simulink model "three_phase_dab"  (R2026a)
settings: Solver=ode23tb  StopTime=param.sim.simlength  FixedStep=tc  MaxStep=param.glb_time.tc
values from neighbouring files (symbols this model uses):
  param = struct()    [init_model.m]
libraries: fl_lib x30, nesl_utility x23, discrete_time_low_pass_filter x6, single_phase_transformer x3, lithium_ion_battery x2, pi_ctrl x2, three_phase_inverter_ideal_switch_based_model x2, three_phase_inverter_mosfet_based_with_thermal_model x2, three_phase_dab_modulator x1
(part 1 of 2)
settings Model: SimulationMode=accelerator  Creator=LTNBDA  LastModifiedBy=dbagn
settings SolverCC: ZeroCrossControl=EnableAll  ZeroCrossAlgorithm=Adaptive  SolverResetMethod=Robust
settings DataIOCC: MaxDataPoints=1  SignalLoggingSaveFormat=ModelDataLogs
settings OptimizationCC: InitFltsAndDblsToZero=on  EfficientMapNaN2IntZero=off
settings DebuggingCC: SaveWithParameterizedLinksMsg=none  SignalResolutionControl=TryResolveAllWithWarning  MultiTaskDSMMsg=warning  MultiTaskCondExecSysMsg=none  MultiTaskRateTransMsg=warning
settings HardwareCC: ProdBitPerLong=64.0  ProdHWDeviceType=Generic->64-bit Embedded Processor (LP64)  TargetBitPerPointer=64.0  TargetBitPerSizeT=64.0  TargetBitPerPtrDiffT=64.0  TargetLongLongMode=on  TargetIntDivRoundTo=Zero  TargetEndianess=LittleEndian  TargetWordSize=64.0  TargetHWDeviceType=MATLAB Host  ProdEqTarget=off
settings SFSimCC: SimCustomHeaderCode=|
  | #include "rpi.h"
  | #include "rpi_simulink.h"
  | #include "mavgflt.h"
  | #include "mavgflt_simulink.h"
  | #include "mavgflts.h"
  | #include "mavgflts_simulink.h"
  | #include "dsmavgflt.h"
  | #include "dsmavgflt_simulink.h"
  | #include "bemf_obsv.h"
  | #include "bemf_obsv_simulink.h"
  | #include "bemf_obsv_load_est.h"
  | #include "bemf_obsv_load_est_simulink.h"
  | #include "dqvector_pi.h"
  | #include "dqvector_pi_simulink.h"
  | #include "sv_pwm_simulink.h"
  | #include "sv_pwm.h"
  | #include "first_harmonic_tracker.h"
  | #include "first_harmonic_tracker_simulink.h"
  | #include "dqpll_thyr.h"
  | #include "dqpll_thyr_simulink.h"
  | #include "dqpll_grid.h"
  | #include "dqpll_grid_simulink.h"
  | #include "linear_double_integrator_observer_simulink.h"
  | #include "linear_double_integrator_observer.h"
  | #include "sv_pwm_cm_simulink.h"
  | #include "sv_pwm_cm.h"
settings SFSimCC: SimUserSources=|
  | "rpi.c"
  | "rpi_simulink.c"
  | "mavgflt_simulink.c"
  | "mavgflt.c"
  | "mavgflts_simulink.c"
  | "mavgflts.c"
  | "dsmavgflt_simulink.c"
  | "dsmavgflt.c"
  | "bemf_obsv_simulink.c"
  | "bemf_obsv.c"
  | "bemf_obsv_load_est_simulink.c"
  | "bemf_obsv_load_est.c"
  | "dqvector_pi.c"
  | "dqvector_pi_simulink.c"
  | "sv_pwm_simulink.c"
  | "sv_pwm.c"
  | "first_harmonic_tracker_simulink.c"
  | "first_harmonic_tracker.c"
  | "dqpll_thyr_simulink.c"
  | "dqpll_thyr.c"
  | "dqpll_grid_simulink.c"
  | "dqpll_grid.c"
  | "linear_double_integrator_observer_simulink.c"
  | "linear_double_integrator_observer.c"
  | "sv_pwm_cm_simulink.c"
  | "sv_pwm_cm.c"
settings SFSimCC: SimUserIncludeDirs=|
  | include
  | src
settings CodeAppCC: MaxIdLength=128.0
settings GRTTargetCC: CombineOutputUpdateFcns=off  GRTInterface=on
settings SimscapeCC: SimscapeNormalizeSystem=off  SimscapeNominalValues="[{\"value\":\"1\",\"unit\":\"A\"},{\"value\":\"1\",\"unit\":\"bar\"},{\"value\":\"1\",\"unit\":\"cm^2\"},{\"value\":\"1\",\"unit\":\"cm^3/s\"},{\"value\":\"1\",\"unit\":\"kJ/kg\"},{\"value\":\"1\",\"unit\":\"kW\"},{\"value\":\"1\",\"unit\":\"l\"},{\"value\":\"1\",\"unit\":\"N\"},{\"value\":\"1\",\"unit\":\"N*m\"},{\"value\":\"1\",\"unit\":\"V\"}]"  SimscapeLogType=none  SimscapeLogDataHistory=5000.0

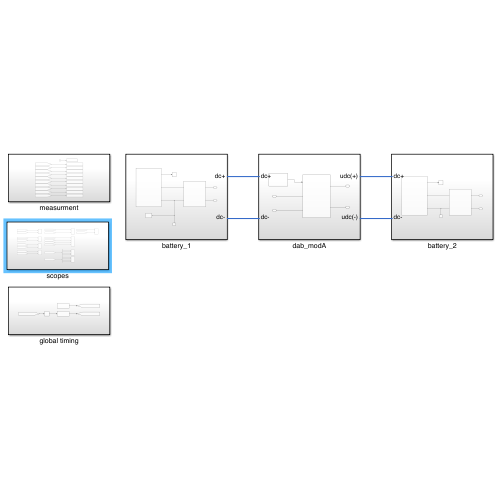
[thumbnail: Simulink's stored preview of the top-level diagram]
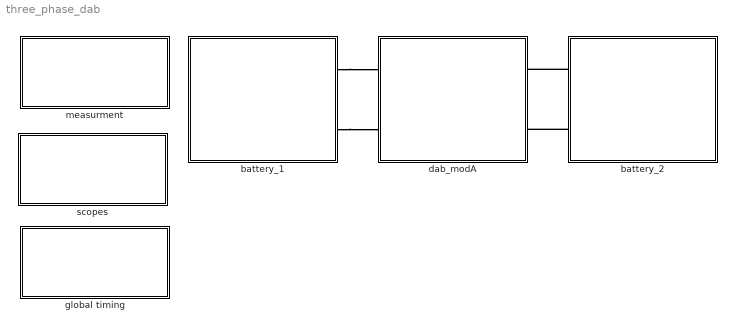
== system three_phase_dab ==
  battery_1 : Subsystem
  battery_2 : Subsystem
  dab_modA : Subsystem
  global timing : Subsystem
  measurment : Subsystem
  scopes : Subsystem
  connections:
  battery_2/RConn2 -- dab_modA/RConn2
  battery_2/RConn1 -- dab_modA/RConn1
  battery_1/RConn1 -- dab_modA/LConn1
  battery_1/RConn2 -- dab_modA/LConn2

== system three_phase_dab/battery_1 ==
  Electrical Reference1 : fl_lib/Electrical/Electrical Elements/Electrical Reference
  Solver Configuration : nesl_utility/Solver Configuration  PhysicalDomain=network_engine_domain  SubClassName=solver  LeftPortType=input  RightPortType=generic  Tones=[]  Harmonics=[]  SimulateNoise=off  Profile=off  UseLocalSampling=off  EnableSwitchedLinearOptims=on  FrequencyDomain=off  UseCCode=off  RelTol=0.001  AbsTol=0.001  MinStep=1e-09  ToWorkspace=off  RevertToSquareIcSolve=off  NumHomotopyIterations=100  PhasorMode=off  PhasorModeNumHarmonics=1  ConsistencySolver=NEWTON_FTOL  CanonicalOrdering=UNORDERED  OptimizeIntermediates=UNOPTIMIZED  IndexReductionMethod=DerivativeReplacement  DoDC=on  ResidualTolerance=1e-3  ConsistencyTolSource=GLOBAL  ConsistencyAbsTol=0.001  ConsistencyRelTol=0.001  ConsistencyTolFactor=0.001  UseLocalSolver=on  LocalSolverChoice=NE_BACKWARD_EULER_ADVANCER  ResolveIndetEquations=on  FunctionEvalNumThread=1  LocalSolverSampleTime=param.glb_time.tc  DoFixedCost=on  MaxNonlinIter=param.sim.nonlinear_iterations  MaxModeIter=2  ComputeImpulses=off  ImpulseIterations=2  LinearAlgebra=auto  LinearAlgebraNumThread=0  EquationFormulation=NE_TIME_EF  DelaysMemoryBudget=1024  AutomaticFiltering=on  FilteringTimeConstant=0.001  PartitionStorageMethod=AS_NEEDED  PartitionMemoryBudget=1024  PartitionMethod=ROBUST  MultibodyUseLocalSolver=off  MultibodyLocalSolverChoice=ODE1  MultibodyLocalSolverSampleTime=0.001
  lithium ion battery 1 : Scope
      settings: ActiveDisplayYMinimum=-6265.3075005586525  ActiveDisplayYMaximum=7146.6490040654116  DataLoggingVariableName=ScopeData3
  lithium_ion_battery : lithium_ion_battery/lithium_ion_battery  Q=param.battery.pack_1.Q  number_of_cells=param.battery.pack_1.number_of_cells  E_1=param.battery.pack_1.E_1  E0=param.battery.pack_1.E0  E1=param.battery.pack_1.E1  E2=param.battery.pack_1.E2  E3=param.battery.pack_1.E3  Elog=param.battery.pack_1.Elog  R0=param.battery.pack_1.R0  R1=param.battery.pack_1.R1  C1=param.battery.pack_1.C1  M=param.battery.pack_1.M  alpha=param.battery.pack_1.alpha  soc_init=param.battery.pack_1.soc_init  ts_battery=param.glb_time.ts_dab  q1Kalman=param.battery.pack_1.q1Kalman  q2Kalman=param.battery.pack_1.q2Kalman  q3Kalman=param.battery.pack_1.q3Kalman  rKalman=param.battery.pack_1.rKalman  tc=param.glb_time.tc  battery_voltage_init_m=param.battery.ocv_1
  single_phase_ui_measure : Subsystem
  dc+ : PMIOPort  Side=Right
  dc- : PMIOPort  Port=2  Side=Right
  wires:
  lithium_ion_battery/1 -> lithium ion battery 1/1
  connections:
  single_phase_ui_measure/LConn2 -- lithium_ion_battery/RConn2 -- Electrical Reference1/LConn1 -- Solver Configuration/RConn1
  single_phase_ui_measure/RConn1 -- dc+/RConn1
  lithium_ion_battery/RConn1 -- single_phase_ui_measure/LConn1
  dc-/RConn1 -- single_phase_ui_measure/RConn2

== system three_phase_dab/battery_2 ==
  Electrical Reference1 : fl_lib/Electrical/Electrical Elements/Electrical Reference
  lithium ion battery 2 : Scope
      settings: ActiveDisplayYMinimum=-4779.68523514888  ActiveDisplayYMaximum=38953.418417165572  DataLoggingVariableName=ScopeData3
  lithium_ion_battery : lithium_ion_battery/lithium_ion_battery  Q=param.battery.pack_2.Q  number_of_cells=param.battery.pack_2.number_of_cells  E_1=param.battery.pack_2.E_1  E0=param.battery.pack_2.E0  E1=param.battery.pack_2.E1  E2=param.battery.pack_2.E2  E3=param.battery.pack_2.E3  Elog=param.battery.pack_2.Elog  R0=param.battery.pack_2.R0  R1=param.battery.pack_2.R1  C1=param.battery.pack_2.C1  M=param.battery.pack_2.M  alpha=param.battery.pack_2.alpha  soc_init=param.battery.pack_2.soc_init  ts_battery=param.glb_time.ts_dab  q1Kalman=param.battery.pack_2.q1Kalman  q2Kalman=param.battery.pack_2.q2Kalman  q3Kalman=param.battery.pack_2.q3Kalman  rKalman=param.battery.pack_2.rKalman  tc=param.glb_time.tc  battery_voltage_init_m=param.battery.ocv_2
  single_phase_ui_measure : Subsystem
  dc+ : PMIOPort  Side=Right
  dc- : PMIOPort  Port=2  Side=Right
  wires:
  lithium_ion_battery/1 -> lithium ion battery 2/1
  connections:
  dc-/RConn1 -- single_phase_ui_measure/RConn2
  lithium_ion_battery/RConn1 -- single_phase_ui_measure/LConn1
  single_phase_ui_measure/RConn1 -- dc+/RConn1
  Electrical Reference1/LConn1 -- lithium_ion_battery/RConn2 -- single_phase_ui_measure/LConn2

== system three_phase_dab/dab_modA ==
  dab_ctrl : Subsystem
  dcdc_with_galvanic_isolation : Subsystem
  udc(+) : PMIOPort  Side=Right
  udc(-) : PMIOPort  Port=2  Side=Right
  dc+ : PMIOPort  Port=3  Side=Left
  dc- : PMIOPort  Port=4  Side=Left
  wires:
  dab_ctrl/1(gate_cmds) -> dcdc_with_galvanic_isolation/1(gate_cmds)
  connections:
  udc(+)/RConn1 -- dcdc_with_galvanic_isolation/RConn1
  udc(-)/RConn1 -- dcdc_with_galvanic_isolation/RConn2
  dc-/RConn1 -- dcdc_with_galvanic_isolation/LConn2
  dc+/RConn1 -- dcdc_with_galvanic_isolation/LConn1

== system three_phase_dab/global timing ==
  Unit Delay : UnitDelay  SampleTime=param.glb_time.tc
  time_afe1 : Subsystem  mask{k=1}
      mask prompts: k "Time Gain"
      mask Display:
      | disp('time-gen');
      | port_label('input', 1, 'crt');
      | port_label('output', 1, 'tout');
  time_afe3 : Subsystem  mask{k=1}
      mask prompts: k "Time Gain"
      mask Display:
      | disp('time-gen');
      | port_label('output', 1, 'tout');
  tag scope: time_dab_module_1=global, time_master=global
  wires:
  time_afe1/1(Out1) -> [time_dab_module_1]
  time_afe3/1(Out1) -> [time_master]
  [local_time_corr_llc_mod1] -> Unit Delay/1
  Unit Delay/1 -> time_afe1/1(correction_time)

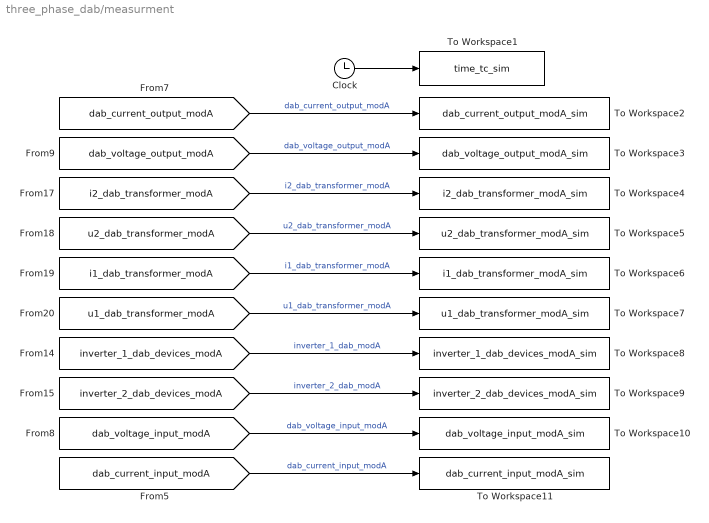
== system three_phase_dab/measurment ==
  Clock : Clock
  To Workspace1 : ToWorkspace  VariableName=time_tc_sim  SampleTime=param.glb_time.tc
      settings: MaxDataPoints=param.glb_time.Nc  Decimation=param.glb_time.decimation_tc
  To Workspace10 : ToWorkspace  VariableName=dab_voltage_input_modA_sim  SampleTime=param.glb_time.tc
      settings: MaxDataPoints=param.glb_time.Nc  Decimation=param.glb_time.decimation_tc
  To Workspace11 : ToWorkspace  VariableName=dab_current_input_modA_sim  SampleTime=param.glb_time.tc
      settings: MaxDataPoints=param.glb_time.Nc  Decimation=param.glb_time.decimation_tc
  To Workspace2 : ToWorkspace  VariableName=dab_current_output_modA_sim  SampleTime=param.glb_time.tc
      settings: MaxDataPoints=param.glb_time.Nc  Decimation=param.glb_time.decimation_tc
  To Workspace3 : ToWorkspace  VariableName=dab_voltage_output_modA_sim  SampleTime=param.glb_time.tc
      settings: MaxDataPoints=param.glb_time.Nc  Decimation=param.glb_time.decimation_tc
  To Workspace4 : ToWorkspace  VariableName=i2_dab_transformer_modA_sim  SampleTime=param.glb_time.tc
      settings: MaxDataPoints=param.glb_time.Nc  Decimation=param.glb_time.decimation_tc
  To Workspace5 : ToWorkspace  VariableName=u2_dab_transformer_modA_sim  SampleTime=param.glb_time.tc
      settings: MaxDataPoints=param.glb_time.Nc  Decimation=param.glb_time.decimation_tc
  To Workspace6 : ToWorkspace  VariableName=i1_dab_transformer_modA_sim  SampleTime=param.glb_time.tc
      settings: MaxDataPoints=param.glb_time.Nc  Decimation=param.glb_time.decimation_tc
  To Workspace7 : ToWorkspace  VariableName=u1_dab_transformer_modA_sim  SampleTime=param.glb_time.tc
      settings: MaxDataPoints=param.glb_time.Nc  Decimation=param.glb_time.decimation_tc
  To Workspace8 : ToWorkspace  VariableName=inverter_1_dab_devices_modA_sim  SampleTime=param.glb_time.tc
      settings: MaxDataPoints=param.glb_time.Nc  Decimation=param.glb_time.decimation_tc
  To Workspace9 : ToWorkspace  VariableName=inverter_2_dab_devices_modA_sim  SampleTime=param.glb_time.tc
      settings: MaxDataPoints=param.glb_time.Nc  Decimation=param.glb_time.decimation_tc
  wires:
  Clock/1 -> To Workspace1/1
  [dab_current_output_modA] -> To Workspace2/1  "dab_current_output_modA"
  [dab_voltage_output_modA] -> To Workspace3/1  "dab_voltage_output_modA"
  [i2_dab_transformer_modA] -> To Workspace4/1  "i2_dab_transformer_modA"
  [u1_dab_transformer_modA] -> To Workspace7/1  "u1_dab_transformer_modA"
  [i1_dab_transformer_modA] -> To Workspace6/1  "i1_dab_transformer_modA"
  [u2_dab_transformer_modA] -> To Workspace5/1  "u2_dab_transformer_modA"
  [inverter_1_dab_devices_modA] -> To Workspace8/1  "inverter_1_dab_modA"
  [inverter_2_dab_devices_modA] -> To Workspace9/1  "inverter_2_dab_modA"
  [dab_voltage_input_modA] -> To Workspace10/1  "dab_voltage_input_modA"
  [dab_current_input_modA] -> To Workspace11/1  "dab_current_input_modA"

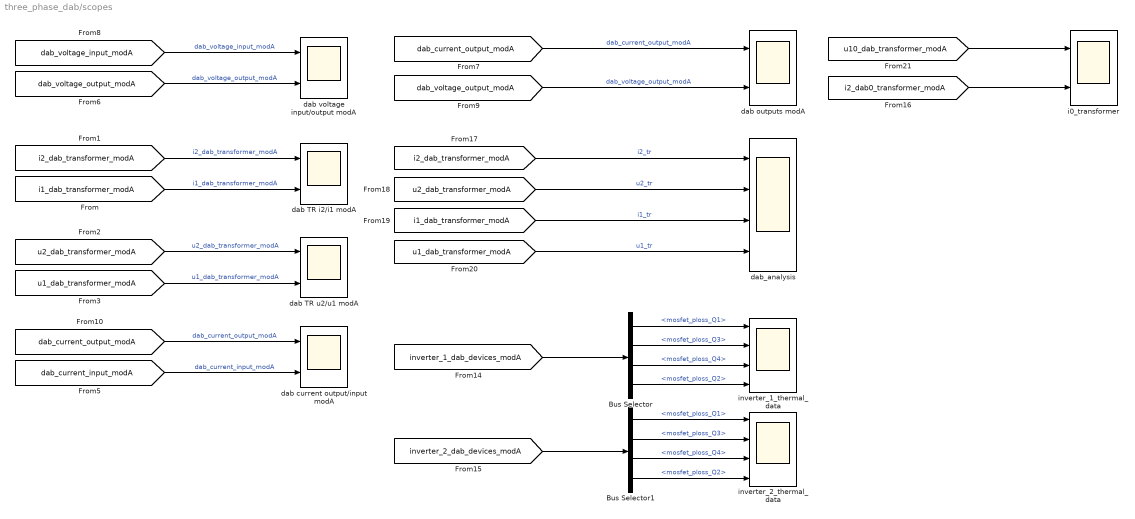
== system three_phase_dab/scopes ==
  Bus Selector : BusSelector  OutputSignals=mosfet_ploss_Q1,mosfet_ploss_Q3,mosfet_ploss_Q4,mosfet_ploss_Q2
  Bus Selector1 : BusSelector  OutputSignals=mosfet_ploss_Q1,mosfet_ploss_Q3,mosfet_ploss_Q4,mosfet_ploss_Q2
  dab TR i2/i1 modA : Scope  NumInputPorts=2
      settings: SampleTime=param.glb_time.tc  ActiveDisplayYMinimum=-2129.3112232140747  ActiveDisplayYMaximum=1620.3891398774613  DataLoggingVariableName=ScopeData13
  dab TR u2/u1 modA : Scope  NumInputPorts=2
      settings: SampleTime=param.glb_time.tc  ActiveDisplayYMinimum=-1578.7453878307324  ActiveDisplayYMaximum=1578.7340154658184  DataLoggingVariableName=ScopeData4
  dab current output/input modA : Scope  NumInputPorts=2
      settings: SampleTime=param.glb_time.tc  ActiveDisplayYMinimum=-1089.9608600530696  ActiveDisplayYMaximum=2070.2962931787843  DataLoggingVariableName=ScopeData8
  dab outputs modA : Scope  NumInputPorts=2
      settings: SampleTime=param.glb_time.tc  ActiveDisplayYMinimum=-644.40009841688664  ActiveDisplayYMaximum=609.5912225853051  DataLoggingVariableName=ScopeData6
  dab voltage input/output modA : Scope  NumInputPorts=2
      settings: SampleTime=param.glb_time.tc  ActiveDisplayYMinimum=1182.800968165963  ActiveDisplayYMaximum=1251.5348190400946  DataLoggingVariableName=ScopeData10
  dab_analysis : Scope  NumInputPorts=4
      settings: ActiveDisplayYMinimum=-934.40964830703967  ActiveDisplayYMaximum=936.03082553931858  DataLoggingVariableName=ScopeData14
  i0_transformer : Scope  NumInputPorts=2
      settings: SampleTime=param.glb_time.tc  ActiveDisplayYMinimum=-1.8947806286936003E-13  ActiveDisplayYMaximum=1.8947806286936003E-13  DataLoggingVariableName=ScopeData11
  inverter_1_thermal_data : Scope  NumInputPorts=4
      settings: SampleTime=param.glb_time.tc  ActiveDisplayYMinimum=-41.459984697896282  ActiveDisplayYMaximum=413.8102017159581
  inverter_2_thermal_data : Scope  NumInputPorts=4
      settings: SampleTime=param.glb_time.tc  ActiveDisplayYMinimum=-81.726801597383641  ActiveDisplayYMaximum=735.5412143764529  DataLoggingVariableName=ScopeData9
  wires:
  [dab_voltage_input_modA] -> dab voltage input/output modA/1  "dab_voltage_input_modA"
  [dab_current_output_modA] -> dab current output/input modA/1  "dab_current_output_modA"
  [dab_voltage_output_modA] -> dab voltage input/output modA/2  "dab_voltage_output_modA"
  [dab_current_input_modA] -> dab current output/input modA/2  "dab_current_input_modA"
  [i2_dab_transformer_modA] -> dab TR i2/i1 modA/1  "i2_dab_transformer_modA"
  [i1_dab_transformer_modA] -> dab TR i2/i1 modA/2  "i1_dab_transformer_modA"
  [u2_dab_transformer_modA] -> dab TR u2/u1 modA/1  "u2_dab_transformer_modA"
  [u1_dab_transformer_modA] -> dab TR u2/u1 modA/2  "u1_dab_transformer_modA"
  [dab_voltage_output_modA] -> dab outputs modA/2  "dab_voltage_output_modA"
  [dab_current_output_modA] -> dab outputs modA/1  "dab_current_output_modA"
  [inverter_1_dab_devices_modA] -> Bus Selector/1
  Bus Selector/1 -> inverter_1_thermal_data/1  "<mosfet_ploss_Q1>"
  Bus Selector/2 -> inverter_1_thermal_data/2  "<mosfet_ploss_Q3>"
  Bus Selector/3 -> inverter_1_thermal_data/3  "<mosfet_ploss_Q4>"
  Bus Selector/4 -> inverter_1_thermal_data/4  "<mosfet_ploss_Q2>"
  Bus Selector1/4 -> inverter_2_thermal_data/4  "<mosfet_ploss_Q2>"
  Bus Selector1/3 -> inverter_2_thermal_data/3  "<mosfet_ploss_Q4>"
  Bus Selector1/2 -> inverter_2_thermal_data/2  "<mosfet_ploss_Q3>"
  Bus Selector1/1 -> inverter_2_thermal_data/1  "<mosfet_ploss_Q1>"
  [inverter_2_dab_devices_modA] -> Bus Selector1/1
  [i2_dab0_transformer_modA] -> i0_transformer/2
  [u10_dab_transformer_modA] -> i0_transformer/1
  [u2_dab_transformer_modA] -> dab_analysis/2  "u2_tr"
  [i2_dab_transformer_modA] -> dab_analysis/1  "i2_tr"
  [u1_dab_transformer_modA] -> dab_analysis/4  "u1_tr"
  [i1_dab_transformer_modA] -> dab_analysis/3  "i1_tr"

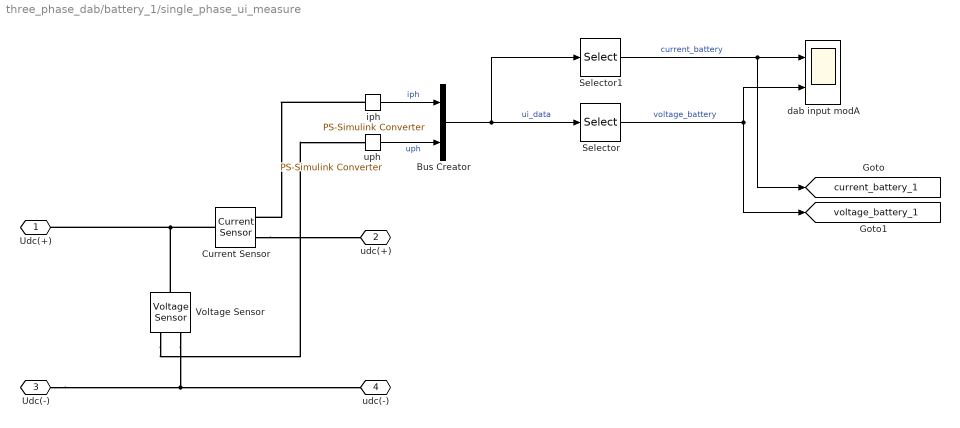
== system three_phase_dab/battery_1/single_phase_ui_measure ==
  Bus Creator : BusCreator  Inputs=2
  Current Sensor : fl_lib/Electrical/Electrical Sensors/Current Sensor
  Selector : Selector  InputPortWidth=2  IndexOptions=Index vector (dialog)  Indices=2  OutputSizes=1
  Selector1 : Selector  InputPortWidth=2  IndexOptions=Index vector (dialog)  Indices=1  OutputSizes=1
  Voltage Sensor : fl_lib/Electrical/Electrical Sensors/Voltage Sensor
  dab input modA : Scope  NumInputPorts=2
      settings: SampleTime=param.glb_time.tc  ActiveDisplayYMinimum=0.011311879178281211  ActiveDisplayYMaximum=0.03131187917828121  DataLoggingVariableName=ScopeData2
  iph : nesl_utility/PS-Simulink Converter  PhysicalDomain=network_engine_domain  SubClassName=ps_output  LeftPortType=input  RightPortType=output  PseudoPeriodic=off  Frequencies=[]  VectorFormat=1-D array  Unit=A  AffineConversion=off
  uph : nesl_utility/PS-Simulink Converter  PhysicalDomain=network_engine_domain  SubClassName=ps_output  LeftPortType=input  RightPortType=output  PseudoPeriodic=off  Frequencies=[]  VectorFormat=1-D array  Unit=V  AffineConversion=off
  Udc(+) : PMIOPort  Side=Left
  udc(+) : PMIOPort  Port=2  Side=Right
  Udc(-) : PMIOPort  Port=3  Side=Left
  udc(-) : PMIOPort  Port=4  Side=Right
  tag scope: current_battery_1=global, voltage_battery_1=global
  wires:
  Bus Creator/1 -> Selector/1, Selector1/1  "ui_data"
  iph/1 -> Bus Creator/1  "iph"
  uph/1 -> Bus Creator/2  "uph"
  Selector1/1 -> [current_battery_1], dab input modA/1  "current_battery"
  Selector/1 -> dab input modA/2, [voltage_battery_1]  "voltage_battery"
  connections:
  iph/LConn1 -- Current Sensor/RConn1
  Voltage Sensor/LConn1 -- Current Sensor/LConn1 -- Udc(+)/RConn1
  Current Sensor/RConn2 -- udc(+)/RConn1
  Voltage Sensor/RConn1 -- uph/LConn1
  Voltage Sensor/RConn2 -- Udc(-)/RConn1 -- udc(-)/RConn1

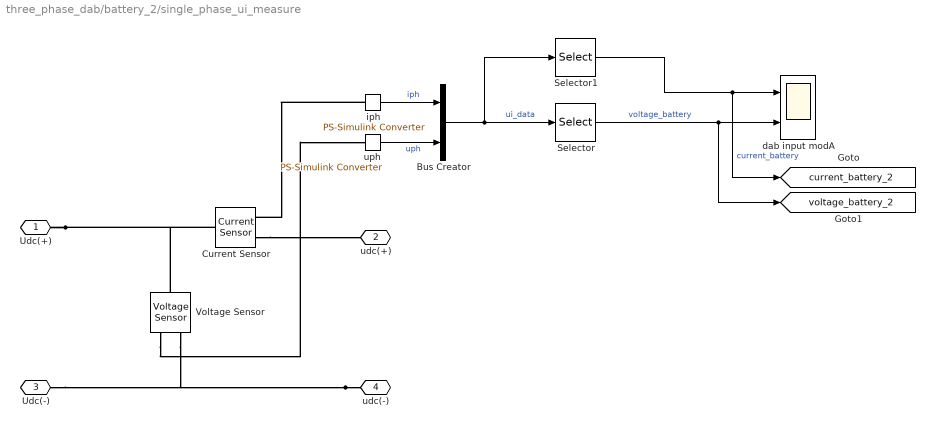
== system three_phase_dab/battery_2/single_phase_ui_measure ==
  Bus Creator : BusCreator  Inputs=2
  Current Sensor : fl_lib/Electrical/Electrical Sensors/Current Sensor
  Selector : Selector  InputPortWidth=2  IndexOptions=Index vector (dialog)  Indices=2  OutputSizes=1
  Selector1 : Selector  InputPortWidth=2  IndexOptions=Index vector (dialog)  Indices=1  OutputSizes=1
  Voltage Sensor : fl_lib/Electrical/Electrical Sensors/Voltage Sensor
  dab input modA : Scope  NumInputPorts=2
      settings: SampleTime=param.glb_time.tc  ActiveDisplayYMinimum=-730.82291169033044  ActiveDisplayYMaximum=-624.34796710988962  DataLoggingVariableName=ScopeData2
  iph : nesl_utility/PS-Simulink Converter  PhysicalDomain=network_engine_domain  SubClassName=ps_output  LeftPortType=input  RightPortType=output  PseudoPeriodic=off  Frequencies=[]  VectorFormat=1-D array  Unit=A  AffineConversion=off
  uph : nesl_utility/PS-Simulink Converter  PhysicalDomain=network_engine_domain  SubClassName=ps_output  LeftPortType=input  RightPortType=output  PseudoPeriodic=off  Frequencies=[]  VectorFormat=1-D array  Unit=V  AffineConversion=off
  Udc(+) : PMIOPort  Side=Left
  udc(+) : PMIOPort  Port=2  Side=Right
  Udc(-) : PMIOPort  Port=3  Side=Left
  udc(-) : PMIOPort  Port=4  Side=Right
  tag scope: current_battery_2=global, voltage_battery_2=global
  wires:
  Selector/1 -> [voltage_battery_2], dab input modA/2  "voltage_battery"
  Selector1/1 -> dab input modA/1, [current_battery_2]  "current_battery"
  uph/1 -> Bus Creator/2  "uph"
  iph/1 -> Bus Creator/1  "iph"
  Bus Creator/1 -> Selector1/1, Selector/1  "ui_data"
  connections:
  udc(-)/RConn1 -- Udc(-)/RConn1 -- Voltage Sensor/RConn2
  Voltage Sensor/RConn1 -- uph/LConn1
  Current Sensor/RConn2 -- udc(+)/RConn1
  Udc(+)/RConn1 -- Current Sensor/LConn1 -- Voltage Sensor/LConn1
  iph/LConn1 -- Current Sensor/RConn1

== system three_phase_dab/dab_modA/dab_ctrl ==
  references1 : Subsystem
  sampling_i_filter2 : Subsystem
  sampling_v_filter3 : Subsystem
  sampling_v_filter4 : Subsystem
  three_phase_dab_modulator : three_phase_dab_modulator/three_phase_dab_modulator  fpwm=param.glb_time.fPWM_DAB  dead_time=param.glb_time.dead_time_DAB  maximum_abs_phase_shift=param.dab3.mod.phi_max  tc=param.glb_time.tc
  ui_ctrl1 : Subsystem
  gate_cmds : Outport
  tag scope: TRGO_DAB_1=global
  wires:
  three_phase_dab_modulator/1 -> [TRGO_DAB_1]
  [TRGO_DAB_1] -> ui_ctrl1/Trigger
  ui_ctrl1/1(phase_displacement) -> three_phase_dab_modulator/2
  three_phase_dab_modulator/2 -> gate_cmds/1
  [time_dab_module_1] -> ui_ctrl1/4(local_time), three_phase_dab_modulator/1
  [dab_current_input_modA] -> sampling_i_filter2/1(in)
  references1/1(vout_ref) -> sampling_v_filter4/1(in)
  [dab_voltage_output_modA] -> sampling_v_filter3/1(in)
  sampling_v_filter3/1(out_pu) -> ui_ctrl1/2(u_pu_dab_output)
  sampling_i_filter2/1(out_pu) -> ui_ctrl1/1(i_pu_dab_input)
  sampling_v_filter4/1(out_pu) -> ui_ctrl1/3(u_pu_dab_output_ref)

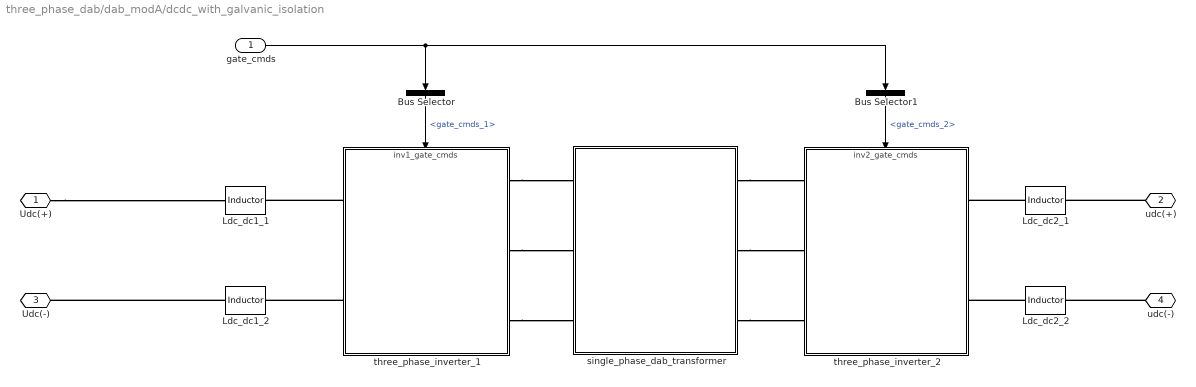
== system three_phase_dab/dab_modA/dcdc_with_galvanic_isolation ==
  gate_cmds : Inport
  Bus Selector : BusSelector  OutputSignals=gate_cmds_1
  Bus Selector1 : BusSelector  OutputSignals=gate_cmds_2
  Ldc_dc1_1 : fl_lib/Electrical/Electrical Elements/Inductor  l=param.dab3.hw.Ldc_dc1/2 H  r=param.dab3.hw.RLdc_dc1/2 Ohm  g=1e-9 1/Ohm  i_specify=off  i_priority=None  i=0 A  i_nominal_specify=off  i_nominal_value=1  i_nominal_unit=A  v_specify=off  v_priority=None  v=0 V  v_nominal_specify=off  v_nominal_value=1  v_nominal_unit=V  i_L_specify=off  i_L_priority=High  i_L=0 A  i_L_nominal_specify=off  i_L_nominal_value=1  i_L_nominal_unit=A
  Ldc_dc1_2 : fl_lib/Electrical/Electrical Elements/Inductor  l=param.dab3.hw.Ldc_dc1/2 H  r=param.dab3.hw.RLdc_dc1/2 Ohm  g=1e-9 1/Ohm  i_specify=off  i_priority=None  i=0 A  i_nominal_specify=off  i_nominal_value=1  i_nominal_unit=A  v_specify=off  v_priority=None  v=0 V  v_nominal_specify=off  v_nominal_value=1  v_nominal_unit=V  i_L_specify=off  i_L_priority=High  i_L=0 A  i_L_nominal_specify=off  i_L_nominal_value=1  i_L_nominal_unit=A
  Ldc_dc2_1 : fl_lib/Electrical/Electrical Elements/Inductor  l=param.dab3.hw.Ldc_dc2/2 H  r=param.dab3.hw.RLdc_dc2/2 Ohm  g=1e-9 1/Ohm  i_specify=off  i_priority=None  i=0 A  i_nominal_specify=off  i_nominal_value=1  i_nominal_unit=A  v_specify=off  v_priority=None  v=0 V  v_nominal_specify=off  v_nominal_value=1  v_nominal_unit=V  i_L_specify=off  i_L_priority=High  i_L=0 A  i_L_nominal_specify=off  i_L_nominal_value=1  i_L_nominal_unit=A
  Ldc_dc2_2 : fl_lib/Electrical/Electrical Elements/Inductor  l=param.dab3.hw.Ldc_dc2/2 H  r=param.dab3.hw.RLdc_dc2/2 Ohm  g=1e-9 1/Ohm  i_specify=off  i_priority=None  i=0 A  i_nominal_specify=off  i_nominal_value=1  i_nominal_unit=A  v_specify=off  v_priority=None  v=0 V  v_nominal_specify=off  v_nominal_value=1  v_nominal_unit=V  i_L_specify=off  i_L_priority=High  i_L=0 A  i_L_nominal_specify=off  i_L_nominal_value=1  i_L_nominal_unit=A
  single_phase_dab_transformer : Subsystem
  three_phase_inverter_1 : Subsystem
      settings: PortSchema="{\"entries\":[{\"content\":{\"sides\":[{\"content\":{\"connectorIds\":[\"LConn1\",\"LConn2\",\"LConn3\"]},\"type\":\"ConnectorPlacement.EquallySpacedRectSide\",\"uuid\":\"c872503a-61af-4937-bdf2-4de4f8645573\"},{\"content\":{\"connectorIds\":[\"RConn1\",\"RConn2\"],\"side\":\"RIGHT\"},\"type\":\"ConnectorPlacement.EquallySpacedRectSide\",\"uuid\":\"3b83f060-86a2-4569-84b5-d9f7c0485347\"},{\"content\":{\"connectorIds\":[\"In1\"],\"side\":\"TOP\"},\"type\":\"ConnectorPlacement.EquallySpacedRectSide\",\"uuid\":\"bf191d46-ce71-4d15-9dd0-24cc57253577\"}]},\"type\":\"ConnectorPlacement.EquallySpacedConnector\",\"uuid\":\"1b28ceee-25d0-45ae-a3c4-c2563f0d63ba\"}],\"packageUris\":[\"http://schema.mathworks.com/mf0/Connector/R2020b\"],\"version\":\"1.0\"}"
  three_phase_inverter_2 : Subsystem
      settings: PortSchema="{\"entries\":[{\"content\":{\"sides\":[{\"content\":{\"connectorIds\":[\"LConn1\",\"LConn2\",\"LConn3\"]},\"type\":\"ConnectorPlacement.EquallySpacedRectSide\",\"uuid\":\"c872503a-61af-4937-bdf2-4de4f8645573\"},{\"content\":{\"connectorIds\":[\"RConn1\",\"RConn2\"],\"side\":\"RIGHT\"},\"type\":\"ConnectorPlacement.EquallySpacedRectSide\",\"uuid\":\"3b83f060-86a2-4569-84b5-d9f7c0485347\"},{\"content\":{\"connectorIds\":[\"In1\"],\"side\":\"TOP\"},\"type\":\"ConnectorPlacement.EquallySpacedRectSide\",\"uuid\":\"bf191d46-ce71-4d15-9dd0-24cc57253577\"}]},\"type\":\"ConnectorPlacement.EquallySpacedConnector\",\"uuid\":\"1b28ceee-25d0-45ae-a3c4-c2563f0d63ba\"}],\"packageUris\":[\"http://schema.mathworks.com/mf0/Connector/R2020b\"],\"version\":\"1.0\"}"
  Udc(+) : PMIOPort  Side=Left
  udc(+) : PMIOPort  Port=2  Side=Right
  Udc(-) : PMIOPort  Port=3  Side=Left
  udc(-) : PMIOPort  Port=4  Side=Right
  wires:
  gate_cmds/1 -> Bus Selector/1, Bus Selector1/1
  Bus Selector/1 -> three_phase_inverter_1/1(inv1_gate_cmds)  "<gate_cmds_1>"
  Bus Selector1/1 -> three_phase_inverter_2/1(inv2_gate_cmds)  "<gate_cmds_2>"
  connections:
  three_phase_inverter_1/RConn1 -- Ldc_dc1_1/RConn1
  udc(-)/RConn1 -- Ldc_dc2_2/RConn1
  Udc(+)/RConn1 -- Ldc_dc1_1/LConn1
  udc(+)/RConn1 -- Ldc_dc2_1/RConn1
  three_phase_inverter_1/LConn1 -- single_phase_dab_transformer/LConn1
  three_phase_inverter_1/LConn2 -- single_phase_dab_transformer/LConn2
  three_phase_inverter_1/LConn3 -- single_phase_dab_transformer/LConn3
  single_phase_dab_transformer/RConn1 -- three_phase_inverter_2/LConn1
  single_phase_dab_transformer/RConn2 -- three_phase_inverter_2/LConn2
  single_phase_dab_transformer/RConn3 -- three_phase_inverter_2/LConn3
  Ldc_dc2_1/LConn1 -- three_phase_inverter_2/RConn1
  three_phase_inverter_1/RConn2 -- Ldc_dc1_2/RConn1
  Ldc_dc1_2/LConn1 -- Udc(-)/RConn1
  Ldc_dc2_2/LConn1 -- three_phase_inverter_2/RConn2

== system three_phase_dab/global timing/time_afe1 ==
  correction_time : Inport
  Constant : Constant
  Gain : Gain  Gain=k
  Product : Product
  Sum : Sum  Inputs=|++
  time_1 : Clock
  Out1 : Outport
  wires:
  time_1/1 -> Gain/1
  Gain/1 -> Product/1
  Product/1 -> Out1/1
  correction_time/1 -> Sum/1
  Sum/1 -> Product/2
  Constant/1 -> Sum/2

== system three_phase_dab/global timing/time_afe3 ==
  Gain : Gain  Gain=k
  time_1 : Clock
  Out1 : Outport
  wires:
  Gain/1 -> Out1/1
  time_1/1 -> Gain/1

== system three_phase_dab/dab_modA/dab_ctrl/references1 ==
  Rate Limiter : RateLimiter  RisingSlewLimit=param.dab3.hw.udc2_nom*10  FallingSlewLimit=-param.dab3.hw.udc2_nom*10  SampleTimeMode=inherited
  Vout_dc_nom : Step  Time=1e-3  FinalValue=param.dab3.hw.udc2_nom  SampleTime=0
  vout_ref : Outport
  wires:
  Rate Limiter/1 -> vout_ref/1
  Vout_dc_nom/1 -> Rate Limiter/1

== system three_phase_dab/dab_modA/dab_ctrl/sampling_i_filter2 ==
  in : Inport
  1/Ti3 : Gain  Gain=1/param.dab3.hw.idc1_bez  OutDataTypeStr=double  SaturateOnIntegerOverflow=on  ParamDataTypeStr=Inherit: Same as input
  out_pu : Outport
  wires:
  in/1 -> 1/Ti3/1
  1/Ti3/1 -> out_pu/1

== system three_phase_dab/dab_modA/dab_ctrl/sampling_v_filter3 ==
  in : Inport
  1/Ti3 : Gain  Gain=1/param.dab3.hw.udc2_bez  OutDataTypeStr=double  SaturateOnIntegerOverflow=on  ParamDataTypeStr=Inherit: Same as input
  out_pu : Outport
  wires:
  in/1 -> 1/Ti3/1
  1/Ti3/1 -> out_pu/1

== system three_phase_dab/dab_modA/dab_ctrl/sampling_v_filter4 ==
  in : Inport
  1/Ti3 : Gain  Gain=1/param.dab3.hw.udc2_bez  OutDataTypeStr=double  SaturateOnIntegerOverflow=on  ParamDataTypeStr=Inherit: Same as input
  Saturation : Saturate  UpperLimit=1  LowerLimit=0  OutDataTypeStr=double
  out_pu : Outport
  wires:
  in/1 -> 1/Ti3/1
  1/Ti3/1 -> Saturation/1
  Saturation/1 -> out_pu/1

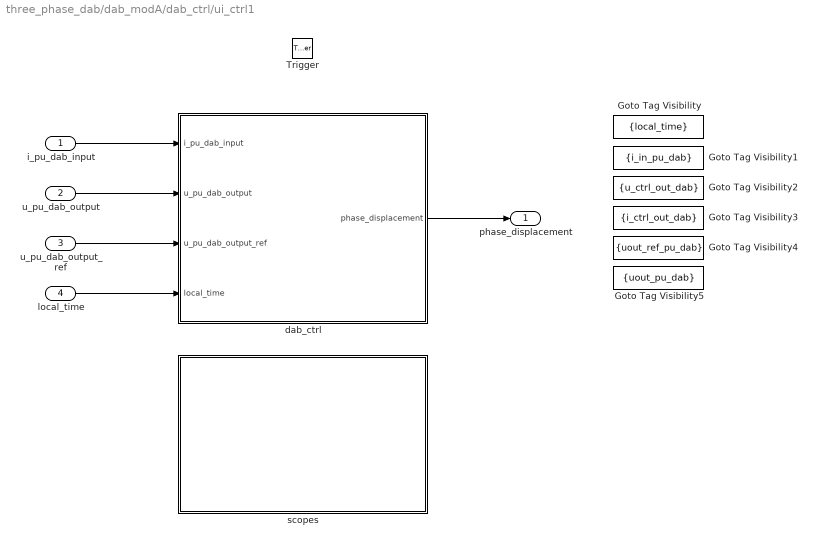
== system three_phase_dab/dab_modA/dab_ctrl/ui_ctrl1 ==
  i_pu_dab_input : Inport
  u_pu_dab_output : Inport  Port=2
  u_pu_dab_output_ref : Inport  Port=3
  local_time : Inport  Port=4
  Trigger : TriggerPort  VariantControl=(inherit)  PortDimensions=1
  Goto Tag Visibility : GotoTagVisibility  GotoTag=local_time
  Goto Tag Visibility1 : GotoTagVisibility  GotoTag=i_in_pu_dab
  Goto Tag Visibility2 : GotoTagVisibility  GotoTag=u_ctrl_out_dab
  Goto Tag Visibility3 : GotoTagVisibility  GotoTag=i_ctrl_out_dab
  Goto Tag Visibility4 : GotoTagVisibility  GotoTag=uout_ref_pu_dab
  Goto Tag Visibility5 : GotoTagVisibility  GotoTag=uout_pu_dab
  dab_ctrl : Subsystem
  scopes : Subsystem
  phase_displacement : Outport
  wires:
  i_pu_dab_input/1 -> dab_ctrl/1(i_pu_dab_input)
  u_pu_dab_output/1 -> dab_ctrl/2(u_pu_dab_output)
  u_pu_dab_output_ref/1 -> dab_ctrl/3(u_pu_dab_output_ref)
  dab_ctrl/1(phase_displacement) -> phase_displacement/1
  local_time/1 -> dab_ctrl/4(local_time)

== system three_phase_dab/dab_modA/dcdc_with_galvanic_isolation/single_phase_dab_transformer ==
  three_phase_hf_transformer : Subsystem
  threephase_vi_measures_stack : Subsystem
  threephase_vi_measures_stack1 : Subsystem
  u1 : PMIOPort  Side=Left
  v1 : PMIOPort  Port=2  Side=Left
  w1 : PMIOPort  Port=3  Side=Left
  u2 : PMIOPort  Port=4  Side=Right
  v2 : PMIOPort  Port=5  Side=Right
  w2 : PMIOPort  Port=6  Side=Right
  connections:
  three_phase_hf_transformer/LConn1 -- threephase_vi_measures_stack/RConn1
  three_phase_hf_transformer/LConn2 -- threephase_vi_measures_stack/RConn2
  three_phase_hf_transformer/LConn3 -- threephase_vi_measures_stack/RConn3
  threephase_vi_measures_stack1/LConn1 -- three_phase_hf_transformer/RConn1
  threephase_vi_measures_stack1/LConn2 -- three_phase_hf_transformer/RConn2
  threephase_vi_measures_stack1/LConn3 -- three_phase_hf_transformer/RConn3
  threephase_vi_measures_stack1/LConn4 -- three_phase_hf_transformer/RConn4
  threephase_vi_measures_stack/RConn4 -- three_phase_hf_transformer/LConn4
  u1/RConn1 -- threephase_vi_measures_stack/LConn1
  v1/RConn1 -- threephase_vi_measures_stack/LConn2
  w1/RConn1 -- threephase_vi_measures_stack/LConn3
  v2/RConn1 -- threephase_vi_measures_stack1/RConn2
  w2/RConn1 -- threephase_vi_measures_stack1/RConn3
  threephase_vi_measures_stack1/RConn1 -- u2/RConn1

== system three_phase_dab/dab_modA/dcdc_with_galvanic_isolation/three_phase_inverter_1 ==
  inv1_gate_cmds : Inport
  dclink_1 : Subsystem
  three_phase_inverter_1 : Subsystem
  u : PMIOPort  Side=Left
  v : PMIOPort  Port=2  Side=Left
  Udc(+) : PMIOPort  Port=3  Side=Right
  Udc(-) : PMIOPort  Port=4  Side=Right
  w : PMIOPort  Port=5  Side=Left
  wires:
  inv1_gate_cmds/1 -> three_phase_inverter_1/1(inv1_gate_cmds)
  connections:
  Udc(+)/RConn1 -- dclink_1/LConn1
  Udc(-)/RConn1 -- dclink_1/LConn2
  dclink_1/RConn1 -- three_phase_inverter_1/LConn1
  three_phase_inverter_1/RConn1 -- u/RConn1
  three_phase_inverter_1/RConn2 -- v/RConn1
  three_phase_inverter_1/LConn2 -- dclink_1/RConn2
  w/RConn1 -- three_phase_inverter_1/RConn3

== system three_phase_dab/dab_modA/dcdc_with_galvanic_isolation/three_phase_inverter_2 ==
  inv2_gate_cmds : Inport
  dclink_2 : Subsystem
  three_phase_inverter_2 : Subsystem
  u : PMIOPort  Side=Left
  v : PMIOPort  Port=2  Side=Left
  udc(+) : PMIOPort  Port=3  Side=Right
  udc(-) : PMIOPort  Port=4  Side=Right
  w : PMIOPort  Port=5  Side=Left
  wires:
  inv2_gate_cmds/1 -> three_phase_inverter_2/1(inv2_gate_cmds)
  connections:
  udc(+)/RConn1 -- dclink_2/RConn1
  udc(-)/RConn1 -- dclink_2/RConn2
  dclink_2/LConn1 -- three_phase_inverter_2/RConn1
  u/RConn1 -- three_phase_inverter_2/LConn1
  v/RConn1 -- three_phase_inverter_2/LConn2
  dclink_2/LConn2 -- three_phase_inverter_2/RConn2
  w/RConn1 -- three_phase_inverter_2/LConn3

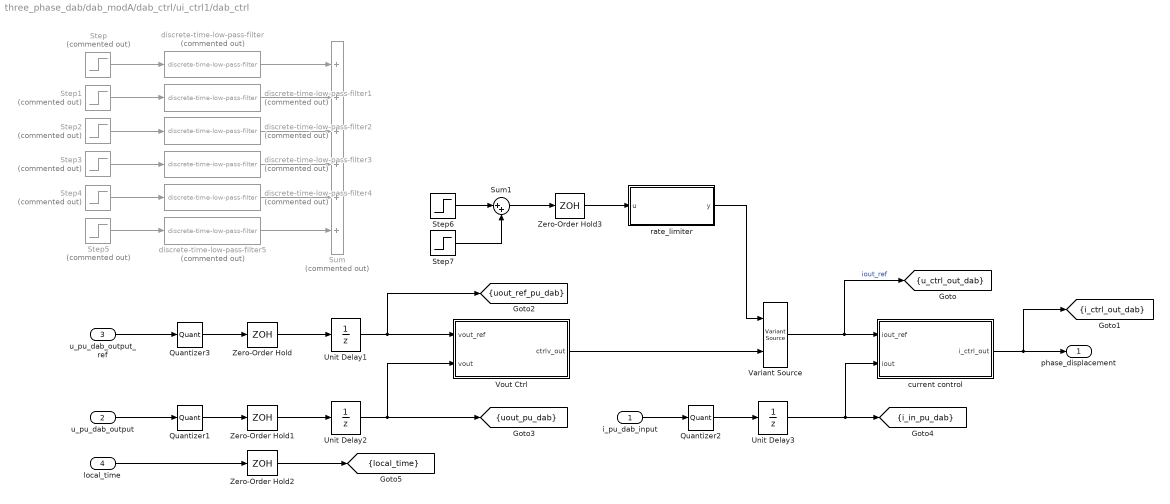
== system three_phase_dab/dab_modA/dab_ctrl/ui_ctrl1/dab_ctrl ==
  i_pu_dab_input : Inport
  u_pu_dab_output : Inport  Port=2
  u_pu_dab_output_ref : Inport  Port=3
  local_time : Inport  Port=4
  Quantizer1 : Quantizer  QuantizationInterval=param.meas.adc12_quantization
  Quantizer2 : Quantizer  QuantizationInterval=param.meas.adc12_quantization
  Quantizer3 : Quantizer  QuantizationInterval=param.meas.adc12_quantization
  Step : Step  Commented=on  Time=0.05  FinalValue=0.25
  Step1 : Step  Commented=on  Time=0.4  FinalValue=0.75
  Step2 : Step  Commented=on  Time=0.6  FinalValue=0.25
  Step3 : Step  Commented=on  Time=0.8  FinalValue=-1
  Step4 : Step  Commented=on  FinalValue=-0.75
  Step5 : Step  Commented=on  Time=1.25  FinalValue=-0.5
  Step6 : Step  Time=param.dab3.bench.t_on  FinalValue=param.dab3.bench.i_ref1
  Step7 : Step  Time=param.dab3.bench.t_rev  FinalValue=param.dab3.bench.i_ref2 - param.dab3.bench.i_ref1
  Sum : Sum  Commented=on  Inputs=++++++
  Sum1 : Sum  Inputs=|++
  Unit Delay1 : UnitDelay  SampleTime=-1
  Unit Delay2 : UnitDelay  SampleTime=-1
  Unit Delay3 : UnitDelay  SampleTime=-1
  Variant Source : VariantSource  VariantControls={true, false}
  Vout Ctrl : Subsystem
  Zero-Order Hold{,1..3} (4 alike) : ZeroOrderHold  SampleTime=-1
  current control : Subsystem
  discrete-time-low-pass-filter{,1..5} (6 alike) : discrete_time_low_pass_filter/discrete-time-low-pass-filter  Commented=on  tau=0.02  ts=param.glb_time.ts_dab
  rate_limiter : Subsystem
  phase_displacement : Outport
  tag scope: i_ctrl_out_dab=scoped, i_in_pu_dab=scoped, local_time=scoped, u_ctrl_out_dab=scoped, uout_pu_dab=scoped, uout_ref_pu_dab=scoped
  wires:
  Vout Ctrl/1(ctrlv_out) -> Variant Source/2
  Variant Source/1 -> [u_ctrl_out_dab], current control/1(iout_ref)  "iout_ref"
  i_pu_dab_input/1 -> Quantizer2/1
  Unit Delay3/1 -> current control/2(iout), [i_in_pu_dab]
  Unit Delay2/1 -> [uout_pu_dab], Vout Ctrl/2(vout)
  Unit Delay1/1 -> Vout Ctrl/1(vout_ref), [uout_ref_pu_dab]
  u_pu_dab_output/1 -> Quantizer1/1
  Step/1 -> discrete-time-low-pass-filter/1
  Step1/1 -> discrete-time-low-pass-filter1/1
  Step2/1 -> discrete-time-low-pass-filter2/1
  Step3/1 -> discrete-time-low-pass-filter3/1
  Step4/1 -> discrete-time-low-pass-filter4/1
  Step5/1 -> discrete-time-low-pass-filter5/1
  discrete-time-low-pass-filter/1 -> Sum/1
  discrete-time-low-pass-filter1/1 -> Sum/2
  discrete-time-low-pass-filter2/1 -> Sum/3
  discrete-time-low-pass-filter3/1 -> Sum/4
  discrete-time-low-pass-filter4/1 -> Sum/5
  discrete-time-low-pass-filter5/1 -> Sum/6
  u_pu_dab_output_ref/1 -> Quantizer3/1
  Quantizer1/1 -> Zero-Order Hold1/1
  Quantizer2/1 -> Unit Delay3/1
  current control/1(i_ctrl_out) -> [i_ctrl_out_dab], phase_displacement/1
  Step6/1 -> Sum1/1
  Step7/1 -> Sum1/2
  Sum1/1 -> Zero-Order Hold3/1
  rate_limiter/1(y) -> Variant Source/1
  Quantizer3/1 -> Zero-Order Hold/1
  Zero-Order Hold/1 -> Unit Delay1/1
  Zero-Order Hold1/1 -> Unit Delay2/1
  local_time/1 -> Zero-Order Hold2/1
  Zero-Order Hold2/1 -> [local_time]
  Zero-Order Hold3/1 -> rate_limiter/1(u)

== system three_phase_dab/dab_modA/dab_ctrl/ui_ctrl1/scopes ==
  Bus Creator : BusCreator  Inputs=2
  Bus Creator1 : BusCreator  Inputs=2
  dab-tracking : Scope  NumInputPorts=2
      settings: ActiveDisplayYMinimum=-25.043212890625  ActiveDisplayYMaximum=28.552978515625  DataLoggingVariableName=ScopeData7
  u_ctrl_out_dab/i_ctrl_out_dab : Scope  NumInputPorts=2
      settings: ActiveDisplayYMinimum=-1.2812486231311795  ActiveDisplayYMaximum=1.531237608180616
  wires:
  Bus Creator1/1 -> dab-tracking/2
  Bus Creator/1 -> dab-tracking/1
  [i_ctrl_out_dab] -> u_ctrl_out_dab/i_ctrl_out_dab/2  "i_ctrl_out_dab"
  [i_in_pu_dab] -> Bus Creator1/2  "i_in_pu_dab"
  [uout_ref_pu_dab] -> Bus Creator/1  "uout_ref_pu_dab"
  [u_ctrl_out_dab] -> u_ctrl_out_dab/i_ctrl_out_dab/1  "u_ctrl_out_dab"
  [u_ctrl_out_dab] -> Bus Creator1/1  "u_ctrl_out_dab"
  [uout_pu_dab] -> Bus Creator/2  "uout_pu_dab"

== system three_phase_dab/dab_modA/dcdc_with_galvanic_isolation/single_phase_dab_transformer/three_phase_hf_transformer ==
  single_phase_transformer : single_phase_transformer/single_phase_transformer  lm_trafo=param.dab3.hw.Lm  m1=param.dab3.hw.n1  m2=param.dab3.hw.n2  rd1_trafo=param.dab3.hw.Rs1  rd2_trafo=param.dab3.hw.Rs2  ld1_trafo=param.dab3.hw.Ld1  ld2_trafo=param.dab3.hw.Ld2  rfe_trafo=param.dab3.hw.Rfe  length_core=param.dab3.hw.core_length  mu0=1.256637e-6  mur=param.dab3.hw.core_mur
  single_phase_transformer1 : single_phase_transformer/single_phase_transformer  lm_trafo=param.dab3.hw.Lm  m1=param.dab3.hw.n1  m2=param.dab3.hw.n2  rd1_trafo=param.dab3.hw.Rs1  rd2_trafo=param.dab3.hw.Rs2  ld1_trafo=param.dab3.hw.Ld1  ld2_trafo=param.dab3.hw.Ld2  rfe_trafo=param.dab3.hw.Rfe  length_core=param.dab3.hw.core_length  mu0=1.256637e-6  mur=param.dab3.hw.core_mur
  single_phase_transformer2 : single_phase_transformer/single_phase_transformer  lm_trafo=param.dab3.hw.Lm  m1=param.dab3.hw.n1  m2=param.dab3.hw.n2  rd1_trafo=param.dab3.hw.Rs1  rd2_trafo=param.dab3.hw.Rs2  ld1_trafo=param.dab3.hw.Ld1  ld2_trafo=param.dab3.hw.Ld2  rfe_trafo=param.dab3.hw.Rfe  length_core=param.dab3.hw.core_length  mu0=1.256637e-6  mur=param.dab3.hw.core_mur
  single_phase_transformer_2: data : Scope
      settings: ActiveDisplayYMinimum=-8112.1514704901265  ActiveDisplayYMaximum=7136.8976315598475  DataLoggingVariableName=ScopeData15
  ua1 : PMIOPort  Side=Left
  ua2 : PMIOPort  Port=2  Side=Right
  ub1 : PMIOPort  Port=3  Side=Left
  ub2 : PMIOPort  Port=4  Side=Right
  uc1 : PMIOPort  Port=5  Side=Left
  uc2 : PMIOPort  Port=6  Side=Right
  un1 : PMIOPort  Port=7  Side=Left
  un2 : PMIOPort  Port=8  Side=Right
  wires:
  single_phase_transformer1/1 -> single_phase_transformer_2: data/1
  connections:
  un2/RConn1 -- single_phase_transformer2/RConn2 -- single_phase_transformer1/RConn2 -- single_phase_transformer/RConn2
  un1/RConn1 -- single_phase_transformer2/LConn2 -- single_phase_transformer1/LConn2 -- single_phase_transformer/LConn2
  single_phase_transformer1/LConn1 -- ub1/RConn1
  single_phase_transformer2/LConn1 -- uc1/RConn1
  single_phase_transformer2/RConn1 -- uc2/RConn1
  single_phase_transformer1/RConn1 -- ub2/RConn1
  single_phase_transformer/RConn1 -- ua2/RConn1
  single_phase_transformer/LConn1 -- ua1/RConn1

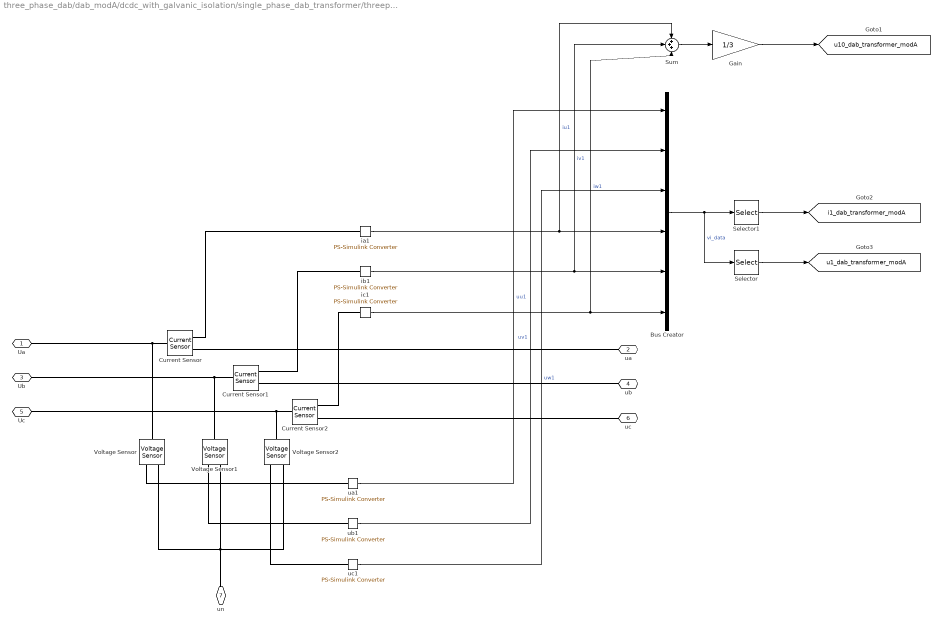
== system three_phase_dab/dab_modA/dcdc_with_galvanic_isolation/single_phase_dab_transformer/threephase_vi_measures_stack ==
  Bus Creator : BusCreator  Inputs=6
  Current Sensor : fl_lib/Electrical/Electrical Sensors/Current Sensor
  Current Sensor1 : fl_lib/Electrical/Electrical Sensors/Current Sensor
  Current Sensor2 : fl_lib/Electrical/Electrical Sensors/Current Sensor
  Gain : Gain  Gain=1/3
  Selector : Selector  InputPortWidth=6  IndexOptions=Index vector (dialog)  Indices=[1 2 3]  OutputSizes=1
  Selector1 : Selector  InputPortWidth=6  IndexOptions=Index vector (dialog)  Indices=[4 5 6]  OutputSizes=1
  Sum : Sum  Inputs=+++
  Voltage Sensor : fl_lib/Electrical/Electrical Sensors/Voltage Sensor
  Voltage Sensor1 : fl_lib/Electrical/Electrical Sensors/Voltage Sensor
  Voltage Sensor2 : fl_lib/Electrical/Electrical Sensors/Voltage Sensor
  ia1 : nesl_utility/PS-Simulink Converter  PhysicalDomain=network_engine_domain  SubClassName=ps_output  LeftPortType=input  RightPortType=output  PseudoPeriodic=off  Frequencies=[]  VectorFormat=1-D array  Unit=A  AffineConversion=off
  ib1 : nesl_utility/PS-Simulink Converter  PhysicalDomain=network_engine_domain  SubClassName=ps_output  LeftPortType=input  RightPortType=output  PseudoPeriodic=off  Frequencies=[]  VectorFormat=1-D array  Unit=A  AffineConversion=off
  ic1 : nesl_utility/PS-Simulink Converter  PhysicalDomain=network_engine_domain  SubClassName=ps_output  LeftPortType=input  RightPortType=output  PseudoPeriodic=off  Frequencies=[]  VectorFormat=1-D array  Unit=A  AffineConversion=off
  ua1 : nesl_utility/PS-Simulink Converter  PhysicalDomain=network_engine_domain  SubClassName=ps_output  LeftPortType=input  RightPortType=output  PseudoPeriodic=off  Frequencies=[]  VectorFormat=1-D array  Unit=V  AffineConversion=off
  ub1 : nesl_utility/PS-Simulink Converter  PhysicalDomain=network_engine_domain  SubClassName=ps_output  LeftPortType=input  RightPortType=output  PseudoPeriodic=off  Frequencies=[]  VectorFormat=1-D array  Unit=V  AffineConversion=off
  uc1 : nesl_utility/PS-Simulink Converter  PhysicalDomain=network_engine_domain  SubClassName=ps_output  LeftPortType=input  RightPortType=output  PseudoPeriodic=off  Frequencies=[]  VectorFormat=1-D array  Unit=V  AffineConversion=off
  Ua : PMIOPort  Side=Left
  ua : PMIOPort  Port=2  Side=Right
  Ub : PMIOPort  Port=3  Side=Left
  ub : PMIOPort  Port=4  Side=Right
  Uc : PMIOPort  Port=5  Side=Left
  uc : PMIOPort  Port=6  Side=Right
  un : PMIOPort  Port=7  Side=Right
  tag scope: i1_dab_transformer_modA=global, u10_dab_transformer_modA=global, u1_dab_transformer_modA=global
  wires:
  Bus Creator/1 -> Selector/1, Selector1/1  "vi_data"
  Selector/1 -> [u1_dab_transformer_modA]
  ib1/1 -> Sum/2, Bus Creator/5  "iv1"
  ia1/1 -> Sum/1, Bus Creator/4  "iu1"
  ic1/1 -> Bus Creator/6, Sum/3  "iw1"
  ua1/1 -> Bus Creator/1  "uu1"
  ub1/1 -> Bus Creator/2  "uv1"
  uc1/1 -> Bus Creator/3  "uw1"
  Selector1/1 -> [i1_dab_transformer_modA]
  Sum/1 -> Gain/1
  Gain/1 -> [u10_dab_transformer_modA]
  connections:
  Current Sensor1/LConn1 -- Ub/RConn1 -- Voltage Sensor1/LConn1
  Voltage Sensor/RConn2 -- un/RConn1 -- Voltage Sensor2/RConn2 -- Voltage Sensor1/RConn2
  Voltage Sensor/RConn1 -- ua1/LConn1
  Current Sensor/RConn2 -- ua/RConn1
  Voltage Sensor1/RConn1 -- ub1/LConn1
  Voltage Sensor2/LConn1 -- Uc/RConn1 -- Current Sensor2/LConn1
  Current Sensor/LConn1 -- Ua/RConn1 -- Voltage Sensor/LConn1
  Current Sensor1/RConn2 -- ub/RConn1
  Voltage Sensor2/RConn1 -- uc1/LConn1
  ib1/LConn1 -- Current Sensor1/RConn1
  ia1/LConn1 -- Current Sensor/RConn1
  ic1/LConn1 -- Current Sensor2/RConn1
  Current Sensor2/RConn2 -- uc/RConn1

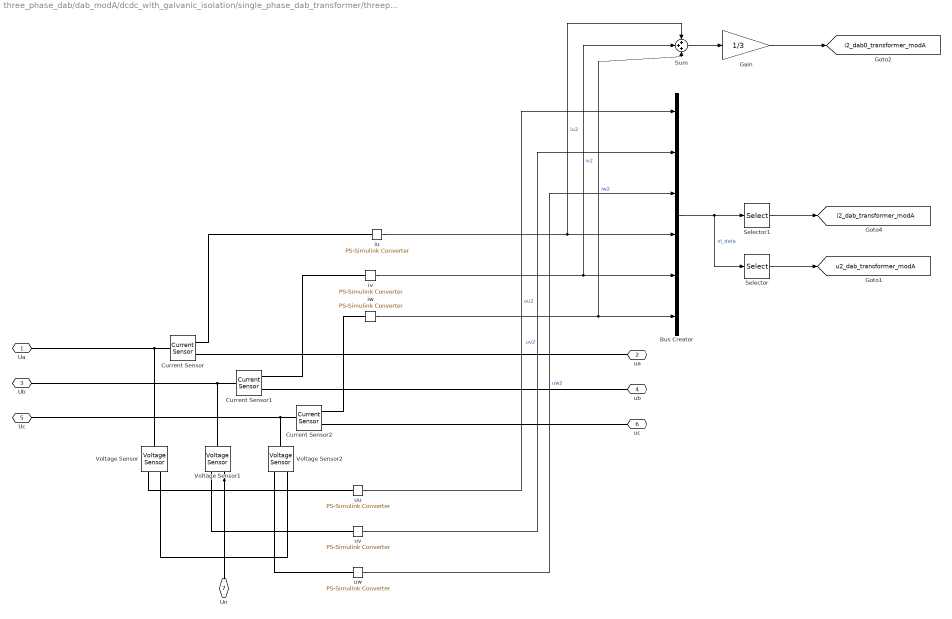
== system three_phase_dab/dab_modA/dcdc_with_galvanic_isolation/single_phase_dab_transformer/threephase_vi_measures_stack1 ==
  Bus Creator : BusCreator  Inputs=6
  Current Sensor : fl_lib/Electrical/Electrical Sensors/Current Sensor
  Current Sensor1 : fl_lib/Electrical/Electrical Sensors/Current Sensor
  Current Sensor2 : fl_lib/Electrical/Electrical Sensors/Current Sensor
  Gain : Gain  Gain=1/3
  Selector : Selector  InputPortWidth=6  IndexOptions=Index vector (dialog)  Indices=[1 2 3]  OutputSizes=1
  Selector1 : Selector  InputPortWidth=6  IndexOptions=Index vector (dialog)  Indices=[4 5 6]  OutputSizes=1
  Sum : Sum  Inputs=+++
  Voltage Sensor : fl_lib/Electrical/Electrical Sensors/Voltage Sensor
  Voltage Sensor1 : fl_lib/Electrical/Electrical Sensors/Voltage Sensor
  Voltage Sensor2 : fl_lib/Electrical/Electrical Sensors/Voltage Sensor
  iu : nesl_utility/PS-Simulink Converter  PhysicalDomain=network_engine_domain  SubClassName=ps_output  LeftPortType=input  RightPortType=output  PseudoPeriodic=off  Frequencies=[]  VectorFormat=1-D array  Unit=A  AffineConversion=off
  iv : nesl_utility/PS-Simulink Converter  PhysicalDomain=network_engine_domain  SubClassName=ps_output  LeftPortType=input  RightPortType=output  PseudoPeriodic=off  Frequencies=[]  VectorFormat=1-D array  Unit=A  AffineConversion=off
  iw : nesl_utility/PS-Simulink Converter  PhysicalDomain=network_engine_domain  SubClassName=ps_output  LeftPortType=input  RightPortType=output  PseudoPeriodic=off  Frequencies=[]  VectorFormat=1-D array  Unit=A  AffineConversion=off
  uu : nesl_utility/PS-Simulink Converter  PhysicalDomain=network_engine_domain  SubClassName=ps_output  LeftPortType=input  RightPortType=output  PseudoPeriodic=off  Frequencies=[]  VectorFormat=1-D array  Unit=V  AffineConversion=off
  uv : nesl_utility/PS-Simulink Converter  PhysicalDomain=network_engine_domain  SubClassName=ps_output  LeftPortType=input  RightPortType=output  PseudoPeriodic=off  Frequencies=[]  VectorFormat=1-D array  Unit=V  AffineConversion=off
  uw : nesl_utility/PS-Simulink Converter  PhysicalDomain=network_engine_domain  SubClassName=ps_output  LeftPortType=input  RightPortType=output  PseudoPeriodic=off  Frequencies=[]  VectorFormat=1-D array  Unit=V  AffineConversion=off
  Ua : PMIOPort  Side=Left
  ua : PMIOPort  Port=2  Side=Right
  Ub : PMIOPort  Port=3  Side=Left
  ub : PMIOPort  Port=4  Side=Right
  Uc : PMIOPort  Port=5  Side=Left
  uc : PMIOPort  Port=6  Side=Right
  Un : PMIOPort  Port=7  Side=Left
  tag scope: i2_dab0_transformer_modA=global, i2_dab_transformer_modA=global, u2_dab_transformer_modA=global
  wires:
  uu/1 -> Bus Creator/1  "uu2"
  Gain/1 -> [i2_dab0_transformer_modA]
  Sum/1 -> Gain/1
  Selector1/1 -> [i2_dab_transformer_modA]
  uw/1 -> Bus Creator/3  "uw2"
  uv/1 -> Bus Creator/2  "uv2"
  iw/1 -> Bus Creator/6, Sum/3  "iw2"
  iu/1 -> Bus Creator/4, Sum/1  "iu2"
  iv/1 -> Bus Creator/5, Sum/2  "iv2"
  Selector/1 -> [u2_dab_transformer_modA]
  Bus Creator/1 -> Selector1/1, Selector/1  "vi_data"
  connections:
  Current Sensor2/RConn2 -- uc/RConn1
  iw/LConn1 -- Current Sensor2/RConn1
  iu/LConn1 -- Current Sensor/RConn1
  iv/LConn1 -- Current Sensor1/RConn1
  Voltage Sensor2/RConn1 -- uw/LConn1
  Current Sensor1/RConn2 -- ub/RConn1
  Voltage Sensor/LConn1 -- Ua/RConn1 -- Current Sensor/LConn1
  Current Sensor2/LConn1 -- Uc/RConn1 -- Voltage Sensor2/LConn1
  Voltage Sensor1/RConn1 -- uv/LConn1
  Current Sensor/RConn2 -- ua/RConn1
  Voltage Sensor/RConn1 -- uu/LConn1
  Voltage Sensor1/RConn2 -- Un/RConn1 -- Voltage Sensor2/RConn2 -- Voltage Sensor/RConn2
  Voltage Sensor1/LConn1 -- Ub/RConn1 -- Current Sensor1/LConn1

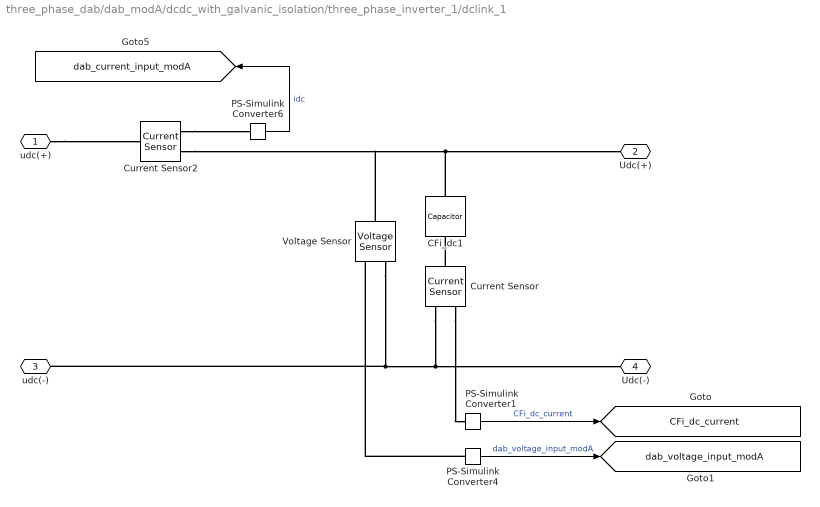
== system three_phase_dab/dab_modA/dcdc_with_galvanic_isolation/three_phase_inverter_1/dclink_1 ==
  CFi_dc1 : fl_lib/Electrical/Electrical Elements/Capacitor  c=param.dab3.hw.Cdc_dc1 F  r=param.dab3.hw.RCdc_dc1 Ohm  g=0 1/Ohm  i_specify=off  i_priority=None  i=0 A  i_nominal_specify=off  i_nominal_value=1  i_nominal_unit=A  v_specify=off  v_priority=None  v=0 V  v_nominal_specify=off  v_nominal_value=1  v_nominal_unit=V  vc_specify=on  vc_priority=High  vc=param.dab3.ic.vc_dc1 V  vc_nominal_specify=off  vc_nominal_value=1  vc_nominal_unit=V
  Current Sensor : fl_lib/Electrical/Electrical Sensors/Current Sensor
  Current Sensor2 : fl_lib/Electrical/Electrical Sensors/Current Sensor
  PS-Simulink Converter1 : nesl_utility/PS-Simulink Converter  PhysicalDomain=network_engine_domain  SubClassName=ps_output  LeftPortType=input  RightPortType=output  PseudoPeriodic=off  Frequencies=[]  VectorFormat=1-D array  Unit=A  AffineConversion=on
  PS-Simulink Converter4 : nesl_utility/PS-Simulink Converter  PhysicalDomain=network_engine_domain  SubClassName=ps_output  LeftPortType=input  RightPortType=output  PseudoPeriodic=off  Frequencies=[]  VectorFormat=1-D array  Unit=V  AffineConversion=on
  PS-Simulink Converter6 : nesl_utility/PS-Simulink Converter  PhysicalDomain=network_engine_domain  SubClassName=ps_output  LeftPortType=input  RightPortType=output  PseudoPeriodic=off  Frequencies=[]  VectorFormat=1-D array  Unit=A  AffineConversion=on
  Voltage Sensor : fl_lib/Electrical/Electrical Sensors/Voltage Sensor
  udc(+) : PMIOPort  Side=Left
  Udc(+) : PMIOPort  Port=2  Side=Right
  udc(-) : PMIOPort  Port=3  Side=Left
  Udc(-) : PMIOPort  Port=4  Side=Right
  tag scope: CFi_dc_current=global, dab_current_input_modA=global, dab_voltage_input_modA=global
  wires:
  PS-Simulink Converter4/1 -> [dab_voltage_input_modA]  "dab_voltage_input_modA"
  PS-Simulink Converter1/1 -> [CFi_dc_current]  "CFi_dc_current"
  PS-Simulink Converter6/1 -> [dab_current_input_modA]  "idc"
  connections:
  Current Sensor/RConn1 -- PS-Simulink Converter1/LConn1
  PS-Simulink Converter4/LConn1 -- Voltage Sensor/RConn1
  Current Sensor/LConn1 -- CFi_dc1/RConn1
  Voltage Sensor/RConn2 -- Current Sensor/RConn2 -- Udc(-)/RConn1 -- udc(-)/RConn1
  CFi_dc1/LConn1 -- Voltage Sensor/LConn1 -- Current Sensor2/RConn2 -- Udc(+)/RConn1
  udc(+)/RConn1 -- Current Sensor2/LConn1
  Current Sensor2/RConn1 -- PS-Simulink Converter6/LConn1
